simulink model "edo"  (R2025b)
settings: Solver=VariableStepAuto  StartTime=0.0  StopTime=10.0  RelTol=1e-3
values from neighbouring files (symbols this model uses):
  Beq = 4.3    [datos.m]
  Bp = 0.0024    [datos.m]
  F = 0    [datos.m]
  g = 9.81    [datos.m]
  I = 0.0079    [datos.m]
  L = 0.3302    [datos.m]
  Mc = 0.7031    [datos.m]
  Mp = 0.23    [datos.m]
settings Model: Creator=Valeria Mar  LastModifiedBy=Valeria Mar

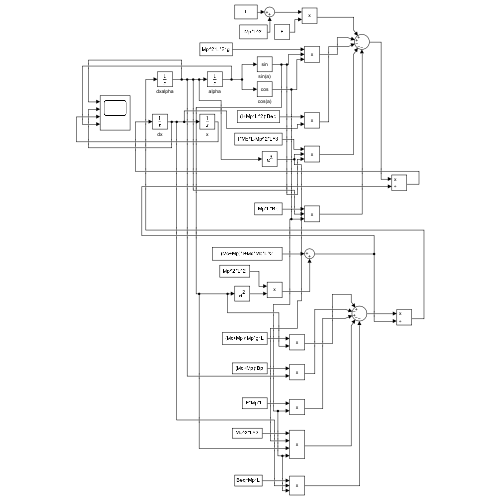
[thumbnail: Simulink's stored preview of the top-level diagram]
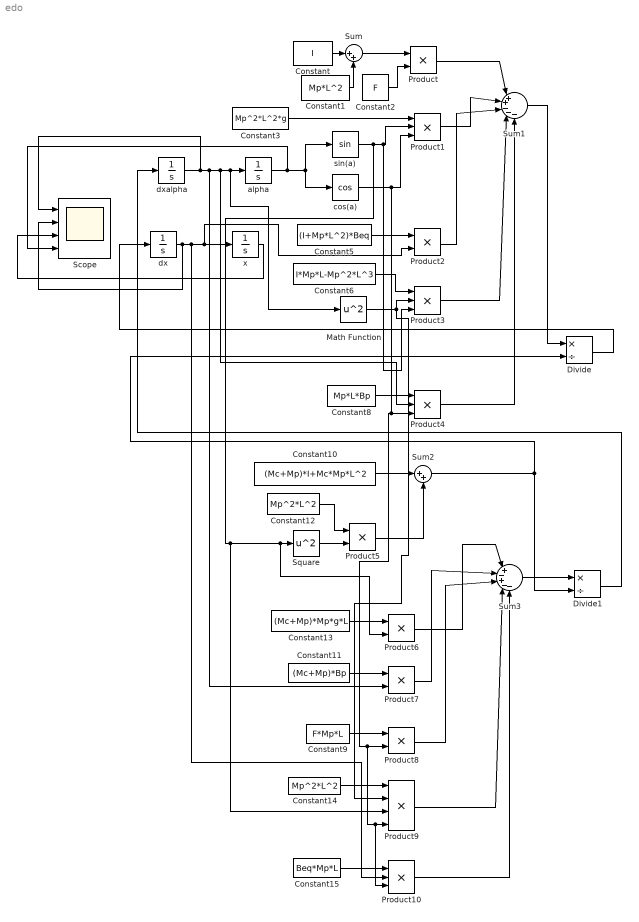
== system edo ==
  Constant : Constant  Value=I
  Constant1 : Constant  Value=Mp*L^2
  Constant10 : Constant  Value=(Mc+Mp)*I+Mc*Mp*L^2
  Constant11 : Constant  Value=(Mc+Mp)*Bp
  Constant12 : Constant  Value=Mp^2*L^2
  Constant13 : Constant  Value=(Mc+Mp)*Mp*g*L
  Constant14 : Constant  Value=Mp^2*L^2
  Constant15 : Constant  Value=Beq*Mp*L  VectorParams1D=off
  Constant2 : Constant  Value=F
  Constant3 : Constant  Value=Mp^2*L^2*g
  Constant5 : Constant  Value=(I+Mp*L^2)*Beq
  Constant6 : Constant  Value=I*Mp*L-Mp^2*L^3
  Constant8 : Constant  Value=Mp*L*Bp
  Constant9 : Constant  Value=F*Mp*L
  Divide : Product  Inputs=*/
  Divide1 : Product  Inputs=*/
  Math Function : Math  Operator=square
  Product{,2,5..8} (6 alike) : Product
  Product{1,3..4,10} (4 alike) : Product  Inputs=3
  Product9 : Product  Inputs=4
  Scope : Scope  NumInputPorts=4
      settings: ActiveDisplayYMinimum=-6.2067981555953793  ActiveDisplayYMaximum=25.280258258050978
  Square : Math  Operator=square
  Sum : Sum  Inputs=|++
  Sum1 : Sum  Inputs=|++---
  Sum2 : Sum  Inputs=|++
  Sum3 : Sum  Inputs=|+-+--
  alpha : Integrator  InitialCondition=1*pi/180
  cos(a) : Trigonometry  Operator=cos
  dx : Integrator
  dxalpha : Integrator
  sin(a) : Trigonometry
  x : Integrator
  wires:
  Constant/1 -> Sum/1
  Sum/1 -> Product/1
  Constant1/1 -> Sum/2
  Constant2/1 -> Product/2
  alpha/1 -> Scope/4, sin(a)/1, cos(a)/1
  Constant3/1 -> Product1/1
  cos(a)/1 -> Product4/3, Product10/3, Product9/4, Product8/2, Product1/3
  Product/1 -> Sum1/1
  Product1/1 -> Sum1/2
  Constant5/1 -> Product2/1
  Product2/1 -> Sum1/3
  Constant6/1 -> Product3/1
  Math Function/1 -> Product9/2, Product3/2
  sin(a)/1 -> Product1/2, Product3/3, Product9/3, Square/1, Product6/2
  Product3/1 -> Sum1/4
  Constant8/1 -> Product4/1
  Product4/1 -> Sum1/5
  Square/1 -> Product5/2
  Constant12/1 -> Product5/1
  Sum1/1 -> Divide/1
  Constant10/1 -> Sum2/1
  Product5/1 -> Sum2/2
  Sum2/1 -> Divide/2, Divide1/2
  Constant13/1 -> Product6/1
  Product6/1 -> Sum3/1
  Constant11/1 -> Product7/1
  Product7/1 -> Sum3/2
  Constant9/1 -> Product8/1
  Product8/1 -> Sum3/3
  Constant14/1 -> Product9/1
  Product9/1 -> Sum3/4
  Constant15/1 -> Product10/1
  Product10/1 -> Sum3/5
  Sum3/1 -> Divide1/1
  dxalpha/1 -> Scope/1, Product7/2, Product4/2, Math Function/1, alpha/1
  dx/1 -> Scope/2, x/1, Product2/2, Product10/2
  Divide/1 -> dx/1
  Divide1/1 -> dxalpha/1
  x/1 -> Scope/3
